simulink model "screeningWorkflow"  (R2026b)
settings: Solver=VariableStepAuto  StopTime=10
settings Model: Creator=azizn  LastModifiedBy=azizn

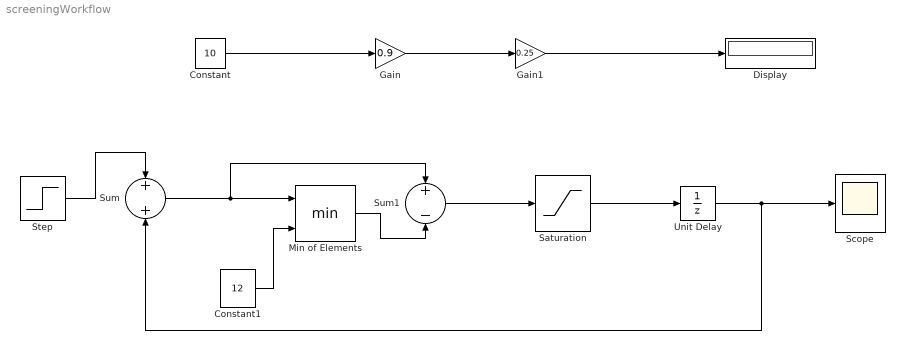
== system screeningWorkflow ==
  Constant : Constant  Value=10
  Constant1 : Constant  Value=12
  Display : Display
  Gain : Gain  Gain=0.9
  Gain1 : Gain  Gain=0.25
  Min of Elements : MinMax  Inputs=2
  Saturation : Saturate  UpperLimit=inf  LowerLimit=0
  Scope : Scope
      settings: MaximizeAxes=On  ActiveDisplayYMinimum=-100.88663112579081  ActiveDisplayYMaximum=40.415970436709287
  Step : Step  Time=5  InitialValue=10  FinalValue=15  SampleTime=0
  Sum : Sum
  Sum1 : Sum  Inputs=+-
  Unit Delay : UnitDelay
  wires:
  Constant/1 -> Gain/1
  Gain/1 -> Gain1/1
  Gain1/1 -> Display/1
  Step/1 -> Sum/1
  Constant1/1 -> Min of Elements/2
  Sum1/1 -> Saturation/1
  Saturation/1 -> Unit Delay/1
  Unit Delay/1 -> Sum/2, Scope/1
  Sum/1 -> Sum1/1, Min of Elements/1
  Min of Elements/1 -> Sum1/2
